simulink subsystem "Integrator_discrete_wrapped_state"  (R2022b)
settings: Solver=VariableStepAuto  StartTime=0.0  StopTime=10.0  RelTol=1e-3
model mask{WrappedStateUpperValue=2*pi, WrappedStateLowerValue=0, x_0=0, T_s=-1}
  mask prompts: WrappedStateUpperValue "Wrapped state upper value"; WrappedStateLowerValue "Wrapped state lower value"; x_0 "Initial state"; T_s "Sample time (-1 for inherited)"
undefined symbols (not defined in the file or in its folder): DiscIntNeverNeededParam
libraries: simulink x2
settings Model: Creator=winkens  LastModifiedBy=winkens
settings SolverCC: AlgebraicLoopSolver=TrustRegion
settings DebuggingCC: UnconnectedInputMsg=warning  UnconnectedOutputMsg=warning  UnconnectedLineMsg=warning  SFMachineParentedDataDiag=warning
settings ModelReferenceCC: EnableRefExpFcnMdlSchedulingChecks=on
settings RTWCC: DLArmComputeVersion=19.05

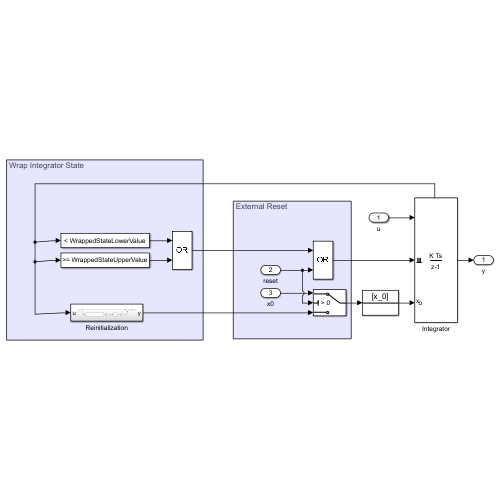
[thumbnail: Simulink's stored preview of the top-level diagram]
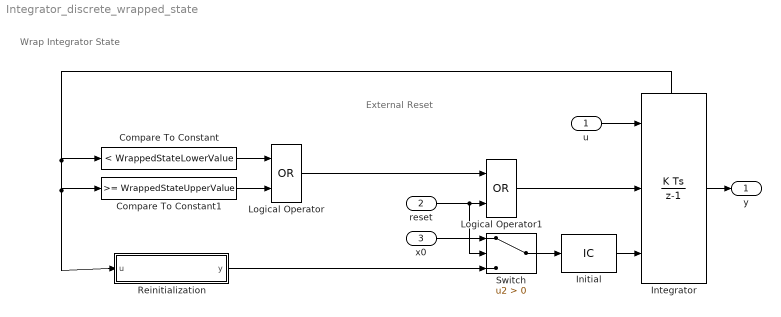
== system Integrator_discrete_wrapped_state ==
  note: External Reset
  note: Wrap Integrator State
  u : Inport
  reset : Inport  Port=2
  x0 : Inport  Port=3
  Compare To Constant : simulink/Logic and Bit Operations/Compare To Constant  relop=<  const=WrappedStateLowerValue  OutDataTypeStr=boolean
  Compare To Constant1 : simulink/Logic and Bit Operations/Compare To Constant  relop=>=  const=WrappedStateUpperValue  OutDataTypeStr=boolean
  Initial : InitialCondition  Value=x_0
  Integrator : DiscreteIntegrator  ExternalReset=sampled level  InitialConditionSource=external  SampleTime=T_s  ShowStatePort=on  ICPrevOutput=DiscIntNeverNeededParam  ICPrevScaledInput=DiscIntNeverNeededParam
  Logical Operator : Logic  Operator=OR  AllPortsSameDT=off  OutDataTypeStr=boolean
  Logical Operator1 : Logic  Operator=OR  AllPortsSameDT=off  OutDataTypeStr=boolean
  Reinitialization : Subsystem
  Switch : Switch  Criteria=u2 > Threshold  SaturateOnIntegerOverflow=off  InputSameDT=off
  y : Outport  VectorParamsAs1DForOutWhenUnconnected=off
  wires:
  Integrator/1 -> y/1
  Compare To Constant1/1 -> Logical Operator/2
  Compare To Constant/1 -> Logical Operator/1
  u/1 -> Integrator/1
  Integrator/State -> Compare To Constant/1, Reinitialization/1(u), Compare To Constant1/1
  Reinitialization/1(y) -> Switch/3
  Logical Operator/1 -> Logical Operator1/1
  Initial/1 -> Integrator/3
  Logical Operator1/1 -> Integrator/2
  reset/1 -> Switch/2, Logical Operator1/2
  x0/1 -> Switch/1
  Switch/1 -> Initial/1

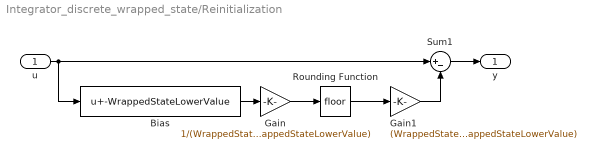
== system Integrator_discrete_wrapped_state/Reinitialization ==
  u : Inport
  Bias : Bias  Bias=-WrappedStateLowerValue  SaturateOnIntegerOverflow=off
  Gain : Gain  Gain=1/(WrappedStateUpperValue-WrappedStateLowerValue)
  Gain1 : Gain  Gain=(WrappedStateUpperValue-WrappedStateLowerValue)
  Rounding Function : Rounding
  Sum1 : Sum  Inputs=|+-
  y : Outport  VectorParamsAs1DForOutWhenUnconnected=off
  wires:
  Sum1/1 -> y/1
  Rounding Function/1 -> Gain1/1
  Bias/1 -> Gain/1
  u/1 -> Bias/1, Sum1/1
  Gain/1 -> Rounding Function/1
  Gain1/1 -> Sum1/2
